simulink model "TB28_A25R_Charging_Stop"  (R2025a)
settings: Solver=FixedStepDiscrete  StartTime=0  StopTime=TB.t_end  FixedStep=TB.dt  RelTol=1e-3
InitFcn:
  | % 모델과 같은 폴더의 초기화 스크립트를 실행해 P(설계 파라미터)와 TB(시험 조건)를 만든다.
  | run(fullfile(fileparts(get_param(bdroot, 'FileName')), 'TB28_init.m'));
values from neighbouring files (symbols this model uses):
  TB = struct()    [TB28_init.m]    (also in run_TB28.m = evalin('base', 'TB'))
libraries: fl_lib x220, nesl_utility x81
(part 1 of 4)
settings Model: Creator=hj000  LastModifiedBy=hj000
settings DataIOCC: SaveOutput=off  SignalLogging=off  SaveTime=off

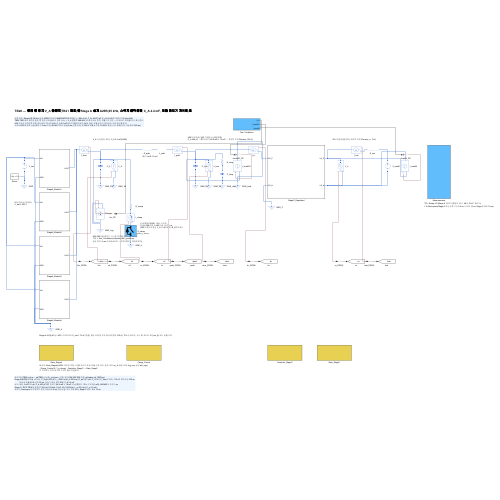
[thumbnail: Simulink's stored preview of the top-level diagram]
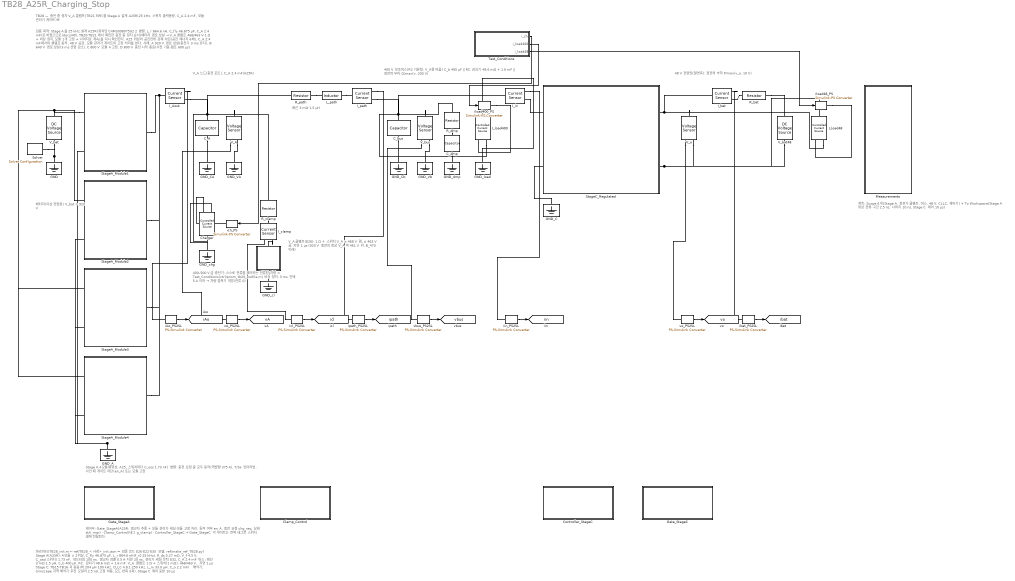
== system TB28_A25R_Charging_Stop ==
  note: TB28 — 충전 중 정지·V_A 클램프(TB21 회로)를 Stage A 설계 A25R(25 kHz, 스위치 출력용량, C_A 2.4 mF, 모듈 관리기 게이트)로
  note: 검증 목적: Stage A를 25 kHz 설계 A25R(위치당 C4MS008075U2 2병렬, L_r 864.6 nH, C_fly 46.875 µF, C_A 2.4 mF)로 바꿨으므로(docs/40),
      | TB20·TB21에서 확인한 충전 중 정지 순서(배터리 경로 상실 → V_A 클램프 468/463 V·1 Ω + 비상 정지, 모듈 1개 고장 → 나머지로 계속)를 다시 확인한다.
      | A25 위상의 공진전류 강제 차단(공진 에너지 6배), C_A 2.4 mF에서의 클램프 동작, 48 V 공급, 모듈 관리기 게이트의 고장 처리를 본다.
      | 사례: A 920 V 경로 상실(충전기 3 ms 유지), B 640 V 경로 상실(3 ms 선형 감소), C 800 V 모듈 4 고장, D 800 V 충전 시작·종료(사전 기동·램프 600 µs)
  note: 배터리(이상 전압원)
      | V_bat = 920 V
  note: V_A 노드(충전 포트), C_A 2.4 mF(A25R)
  note: 400–500 V급 충전기: 스스로 전류를 제어하는 전류원
      | 지령 = Test_Conditions(ctrl/prism_tb20_profile.m)
      | 비상 정지: 3 ms 안에 5 A 이하 → 차량 접촉기 개방(전류 0)
  note: V_A 클램프(E26): 1 Ω + 스위치
      | V_A ≥ 468 V 켬, ≤ 463 V 끔, 지연 1 µs
      | (920 V 충전의 정상 V_A 약 461 V 위, B_470 아래)
  note: Stage A 4모듈(8위상, A25, 스위치마다 C_oss 1.73 nF) 병렬: 충전 요청 중 모두 동작(역방향 375 A), T/16 인터리빙. 사건 때 게이트 차단(en_A) 또는 모듈 고장
  note: 배선 3 mΩ·1.5 µH
  note: 400 V 보조버스(R2 기본형: V_A를 따름)
      | C_b 400 µF ∥ RC 감쇠기 48.6 mΩ + 1.6 mF ∥ 정전력 부하 Q/max(v, 200 V)
  note: 48 V 전원망(절연측): 정전력 부하 P/max(v_o, 10 V)
  note: 제어부: Gate_StageA(A25R: 영교차 추종 + 모듈 관리기·셰딩·모듈 고장 처리, 동작 여부 en_A, 충전 요청 chg_req, 상태 stA_mgr)
      | · Clamp_Control(태그 g_clamp) · Controller_StageC → Gate_StageC
      | 각 게이트는 전역 태그로 스위치 셀에 전달된다.
  note: 계측: Scope 6개(Stage A, 충전기·클램프, 버스, 48 V, CLLC, 제어기)
      | + To Workspace(Stage A 위상 전류·구간 2.5 ns, 나머지 10 ns, Stage C 제어 10 µs)
  note: 파라미터(TB28_init.m ← ref/TB28_<사례>_init.json = 검증 코드 E26·E22·E35 모델, ref/make_ref_TB28.py)
      | Stage A(A25R): 4모듈 × 2위상, C_fly 46.875 µF, L_r 864.6 nH(f_r0 25 kHz), R_ds 5.27 mΩ, V_f 4.5 V, C_oss(스위치) 1.73 nF, 데드타임 100 ns,
      |          영교차 검출 0.5 A·지연 20 ns, 관리기·셰딩 문턱 E32, C_A 2.4 mF
      | 버스: 배선 3 mΩ·1.5 µH, C_b 400 µF, RC 감쇠기 48.6 mΩ + 1.6 mF. V_A 클램프 1 Ω + 스위치(1 mΩ), 468/463 V, 지연 1 µs
      | Stage C: TB15·TB16과 같음(벅 204 µH·100 kHz, CLLC 4.8:1·250 kHz, L_m 33.0 µH, C_o 2.2 mF)
      | 해석기: Simscape 지역 해석기 후진 오일러 2.5 ns(고정 비용, 모드 반복 3회), Stage C 제어 표본 10 µs
  C_A : fl_lib/Electrical/Electrical Elements/Capacitor  c=TB.A.CA F  r=1e-6 Ohm  g=0 1/Ohm  i_specify=off  i_priority=None  i=0 A  i_nominal_specify=off  i_nominal_value=1  i_nominal_unit=A  v_specify=off  v_priority=None  v=0 V  v_nominal_specify=off  v_nominal_value=1  v_nominal_unit=V  vc_specify=on  vc_priority=High  vc=TB.vA0 V  vc_nominal_specify=off  vc_nominal_value=1  vc_nominal_unit=V
  C_bus : fl_lib/Electrical/Electrical Elements/Capacitor  c=TB.Cb F  r=1e-6 Ohm  g=0 1/Ohm  i_specify=off  i_priority=None  i=0 A  i_nominal_specify=off  i_nominal_value=1  i_nominal_unit=A  v_specify=off  v_priority=None  v=0 V  v_nominal_specify=off  v_nominal_value=1  v_nominal_unit=V  vc_specify=on  vc_priority=High  vc=TB.vb0 V  vc_nominal_specify=off  vc_nominal_value=1  vc_nominal_unit=V
  C_dmp : fl_lib/Electrical/Electrical Elements/Capacitor  c=TB.Cdmp F  r=1e-6 Ohm  g=0 1/Ohm  i_specify=off  i_priority=None  i=0 A  i_nominal_specify=off  i_nominal_value=1  i_nominal_unit=A  v_specify=off  v_priority=None  v=0 V  v_nominal_specify=off  v_nominal_value=1  v_nominal_unit=V  vc_specify=on  vc_priority=High  vc=TB.vb0 V  vc_nominal_specify=off  vc_nominal_value=1  vc_nominal_unit=V
  Charger : fl_lib/Electrical/Electrical Sources/Controlled Current Source
  Clamp_Control : Subsystem
  Controller_StageC : Subsystem
  GND : fl_lib/Electrical/Electrical Elements/Electrical Reference
  GND_A : fl_lib/Electrical/Electrical Elements/Electrical Reference
  GND_C : fl_lib/Electrical/Electrical Elements/Electrical Reference
  GND_CA : fl_lib/Electrical/Electrical Elements/Electrical Reference
  GND_Cb : fl_lib/Electrical/Electrical Elements/Electrical Reference
  GND_VA : fl_lib/Electrical/Electrical Elements/Electrical Reference
  GND_Vb : fl_lib/Electrical/Electrical Elements/Electrical Reference
  GND_chg : fl_lib/Electrical/Electrical Elements/Electrical Reference
  GND_cl : fl_lib/Electrical/Electrical Elements/Electrical Reference
  GND_dmp : fl_lib/Electrical/Electrical Elements/Electrical Reference
  GND_load : fl_lib/Electrical/Electrical Elements/Electrical Reference
  Gate_StageA : Subsystem
  Gate_StageC : Subsystem
  I_Aout : fl_lib/Electrical/Electrical Sensors/Current Sensor
  I_bat : fl_lib/Electrical/Electrical Sensors/Current Sensor
  I_clamp : fl_lib/Electrical/Electrical Sensors/Current Sensor
  I_in : fl_lib/Electrical/Electrical Sensors/Current Sensor
  I_load400 : fl_lib/Electrical/Electrical Sources/Controlled Current Source
  I_load48 : fl_lib/Electrical/Electrical Sources/Controlled Current Source
  I_path : fl_lib/Electrical/Electrical Sensors/Current Sensor
  L_path : fl_lib/Electrical/Electrical Elements/Inductor  l=TB.Lpath H  r=0 Ohm  g=1e-9 1/Ohm  i_specify=off  i_priority=None  i=0 A  i_nominal_specify=off  i_nominal_value=1  i_nominal_unit=A  v_specify=off  v_priority=None  v=0 V  v_nominal_specify=off  v_nominal_value=1  v_nominal_unit=V  i_L_specify=on  i_L_priority=High  i_L=TB.iw0 A  i_L_nominal_specify=off  i_L_nominal_value=1  i_L_nominal_unit=A
  Measurements : Subsystem
  R_bat : fl_lib/Electrical/Electrical Elements/Resistor  R=TB.Rbat Ohm  i_specify=off  i_priority=None  i=0 A  i_nominal_specify=off  i_nominal_value=1  i_nominal_unit=A  v_specify=off  v_priority=None  v=0 V  v_nominal_specify=off  v_nominal_value=1  v_nominal_unit=V
  R_clamp : fl_lib/Electrical/Electrical Elements/Resistor  R=TB.Rclamp Ohm  i_specify=off  i_priority=None  i=0 A  i_nominal_specify=off  i_nominal_value=1  i_nominal_unit=A  v_specify=off  v_priority=None  v=0 V  v_nominal_specify=off  v_nominal_value=1  v_nominal_unit=V
  R_dmp : fl_lib/Electrical/Electrical Elements/Resistor  R=TB.Rdmp Ohm  i_specify=off  i_priority=None  i=0 A  i_nominal_specify=off  i_nominal_value=1  i_nominal_unit=A  v_specify=off  v_priority=None  v=0 V  v_nominal_specify=off  v_nominal_value=1  v_nominal_unit=V
  R_path : fl_lib/Electrical/Electrical Elements/Resistor  R=TB.Rpath Ohm  i_specify=off  i_priority=None  i=0 A  i_nominal_specify=off  i_nominal_value=1  i_nominal_unit=A  v_specify=off  v_priority=None  v=0 V  v_nominal_specify=off  v_nominal_value=1  v_nominal_unit=V
  S_clamp : Subsystem  mask(PRISM-Hub switch cell){Ron=1e-3, Goff=1e-8, Vf=2, Rd=1e-3, Goffd=1e-8}
      mask prompts: Ron "도통 저항 R_on [Ohm]"; Goff "차단 컨덕턴스 G_off [S]"; Vf "다이오드 순방향 전압 Vf [V]"; Rd "다이오드 도통 저항 R_d [Ohm]"; Goffd "다이오드 차단 컨덕턴스 [S]"
      mask help: 전력 반도체 스위치 셀 S_clamp. 게이트 태그 g_clamp.
      settings: AttributesFormatString=gate: g_clamp
      mask Display:
      | plot([0.50 0.50 ],[0.95 0.65 ],[0.50 0.74 ],[0.65 0.35 ],[0.50 0.50 ],[0.35 0.05 ]);
      | plot([0.50 0.20 0.20 ],[0.80 0.80 0.58 ],[0.20 0.20 0.50 ],[0.42 0.20 0.20 ]);
      | plot([0.20 0.10 0.30 0.20 ],[0.58 0.42 0.42 0.58 ],[0.10 0.30 ],[0.58 0.58 ]);
      | port_label('LConn',1,'D');
      | port_label('RConn',1,'S');
  Solver : nesl_utility/Solver Configuration  PhysicalDomain=network_engine_domain  SubClassName=solver  LeftPortType=input  RightPortType=generic  Tones=[]  Harmonics=[]  SimulateNoise=off  Profile=off  UseLocalSampling=off  EnableSwitchedLinearOptims=on  FrequencyDomain=off  UseCCode=off  RelTol=0.001  AbsTol=0.001  MinStep=1e-09  ToWorkspace=off  RevertToSquareIcSolve=off  NumHomotopyIterations=100  PhasorMode=off  PhasorModeNumHarmonics=1  ConsistencySolver=NEWTON_XTOL_AFTER_FTOL  IndexReductionMethod=DerivativeReplacement  DoDC=off  ResidualTolerance=1e-9  ConsistencyTolSource=GLOBAL  ConsistencyAbsTol=0.001  ConsistencyRelTol=0.001  ConsistencyTolFactor=0.001  UseLocalSolver=on  LocalSolverChoice=NE_BACKWARD_EULER_ADVANCER  ResolveIndetEquations=on  FunctionEvalNumThread=1  LocalSolverSampleTime=TB.dt  DoFixedCost=on  MaxNonlinIter=3  MaxModeIter=2  ComputeImpulses=off  ImpulseIterations=2  LinearAlgebra=auto  LinearAlgebraNumThread=0  EquationFormulation=NE_TIME_EF  DelaysMemoryBudget=1024  AutomaticFiltering=on  FilteringTimeConstant=0.001  PartitionStorageMethod=AS_NEEDED  PartitionMemoryBudget=1024  PartitionMethod=ROBUST  MultibodyUseLocalSolver=off  MultibodyLocalSolverChoice=ODE1  MultibodyLocalSolverSampleTime=0.001
  StageA_Module1 : Subsystem
  StageA_Module2 : Subsystem
  StageA_Module3 : Subsystem
  StageA_Module4 : Subsystem
  StageC_Regulated : Subsystem
  Test_Conditions : Subsystem
  V_A : fl_lib/Electrical/Electrical Sensors/Voltage Sensor
  V_bat : fl_lib/Electrical/Electrical Sources/DC Voltage Source  v0=TB.vbat V
  V_bat48 : fl_lib/Electrical/Electrical Sources/DC Voltage Source  v0=TB.OCV V
  V_bus : fl_lib/Electrical/Electrical Sensors/Voltage Sensor
  V_o : fl_lib/Electrical/Electrical Sensors/Voltage Sensor
  iAo_PS2SL : nesl_utility/PS-Simulink Converter  PhysicalDomain=network_engine_domain  SubClassName=ps_output  LeftPortType=input  RightPortType=output  PseudoPeriodic=off  Frequencies=[]  VectorFormat=inherit  Unit=inherit  AffineConversion=off
  ibat_PS2SL : nesl_utility/PS-Simulink Converter  PhysicalDomain=network_engine_domain  SubClassName=ps_output  LeftPortType=input  RightPortType=output  PseudoPeriodic=off  Frequencies=[]  VectorFormat=inherit  Unit=inherit  AffineConversion=off
  ich_PS : nesl_utility/Simulink-PS Converter  PhysicalDomain=network_engine_domain  SubClassName=ps_input  LeftPortType=input  RightPortType=output  PseudoPeriodic=off  Frequencies=[]  NoiseDistribution=none  NoiseParameters=[]  Unit=1  AffineConversion=off  FilteringAndDerivatives=provide  SimscapeFilterOrder=1  InputFilterTimeConstant=0.001  UdotUserProvided=0
  icl_PS2SL : nesl_utility/PS-Simulink Converter  PhysicalDomain=network_engine_domain  SubClassName=ps_output  LeftPortType=input  RightPortType=output  PseudoPeriodic=off  Frequencies=[]  VectorFormat=inherit  Unit=inherit  AffineConversion=off
  iin_PS2SL : nesl_utility/PS-Simulink Converter  PhysicalDomain=network_engine_domain  SubClassName=ps_output  LeftPortType=input  RightPortType=output  PseudoPeriodic=off  Frequencies=[]  VectorFormat=inherit  Unit=inherit  AffineConversion=off
  iload400_PS : nesl_utility/Simulink-PS Converter  PhysicalDomain=network_engine_domain  SubClassName=ps_input  LeftPortType=input  RightPortType=output  PseudoPeriodic=off  Frequencies=[]  NoiseDistribution=none  NoiseParameters=[]  Unit=1  AffineConversion=off  FilteringAndDerivatives=provide  SimscapeFilterOrder=1  InputFilterTimeConstant=0.001  UdotUserProvided=0
  iload48_PS : nesl_utility/Simulink-PS Converter  PhysicalDomain=network_engine_domain  SubClassName=ps_input  LeftPortType=input  RightPortType=output  PseudoPeriodic=off  Frequencies=[]  NoiseDistribution=none  NoiseParameters=[]  Unit=1  AffineConversion=off  FilteringAndDerivatives=provide  SimscapeFilterOrder=1  InputFilterTimeConstant=0.001  UdotUserProvided=0
  ipath_PS2SL : nesl_utility/PS-Simulink Converter  PhysicalDomain=network_engine_domain  SubClassName=ps_output  LeftPortType=input  RightPortType=output  PseudoPeriodic=off  Frequencies=[]  VectorFormat=inherit  Unit=inherit  AffineConversion=off
  vA_PS2SL : nesl_utility/PS-Simulink Converter  PhysicalDomain=network_engine_domain  SubClassName=ps_output  LeftPortType=input  RightPortType=output  PseudoPeriodic=off  Frequencies=[]  VectorFormat=inherit  Unit=inherit  AffineConversion=off
  vbus_PS2SL : nesl_utility/PS-Simulink Converter  PhysicalDomain=network_engine_domain  SubClassName=ps_output  LeftPortType=input  RightPortType=output  PseudoPeriodic=off  Frequencies=[]  VectorFormat=inherit  Unit=inherit  AffineConversion=off
  vo_PS2SL : nesl_utility/PS-Simulink Converter  PhysicalDomain=network_engine_domain  SubClassName=ps_output  LeftPortType=input  RightPortType=output  PseudoPeriodic=off  Frequencies=[]  VectorFormat=inherit  Unit=inherit  AffineConversion=off
  tag scope: iAo=global, ibat=global, icl=global, iin=global, ipath=global, vA=global, vbus=global, vo=global
  wires:
  iAo_PS2SL/1 -> [iAo]
  vA_PS2SL/1 -> [vA]
  icl_PS2SL/1 -> [icl]
  ipath_PS2SL/1 -> [ipath]
  vbus_PS2SL/1 -> [vbus]
  iin_PS2SL/1 -> [iin]
  vo_PS2SL/1 -> [vo]
  ibat_PS2SL/1 -> [ibat]
  Test_Conditions/1(i_ch) -> ich_PS/1
  Test_Conditions/2(i_load400) -> iload400_PS/1
  Test_Conditions/3(i_load48) -> iload48_PS/1
  connections:
  GND/LConn1 -- Solver/RConn1 -- V_bat/RConn1
  StageA_Module1/LConn1 -- V_bat/LConn1 -- StageA_Module2/LConn1 -- StageA_Module3/LConn1 -- StageA_Module4/LConn1
  StageA_Module1/LConn2 -- StageA_Module2/LConn2 -- StageA_Module3/LConn2 -- GND_A/LConn1 -- StageA_Module4/LConn2
  StageA_Module1/RConn1 -- StageA_Module2/RConn1 -- StageA_Module3/RConn1 -- I_Aout/LConn1 -- StageA_Module4/RConn1
  I_Aout/RConn2 -- V_A/LConn1 -- Charger/LConn1 -- R_clamp/LConn1 -- C_A/LConn1 -- R_path/LConn1
  C_A/RConn1 -- GND_CA/LConn1
  V_A/RConn2 -- GND_VA/LConn1
  Charger/RConn2 -- GND_chg/LConn1
  ich_PS/RConn1 -- Charger/RConn1
  R_clamp/RConn1 -- I_clamp/LConn1
  I_clamp/RConn2 -- S_clamp/LConn1
  S_clamp/RConn1 -- GND_cl/LConn1
  R_path/RConn1 -- L_path/LConn1
  L_path/RConn1 -- I_path/LConn1
  I_path/RConn2 -- V_bus/LConn1 -- R_dmp/LConn1 -- I_load400/RConn2 -- C_bus/LConn1 -- I_in/LConn1
  C_bus/RConn1 -- GND_Cb/LConn1
  V_bus/RConn2 -- GND_Vb/LConn1
  R_dmp/RConn1 -- C_dmp/LConn1
  C_dmp/RConn1 -- GND_dmp/LConn1
  I_load400/LConn1 -- GND_load/LConn1
  iload400_PS/RConn1 -- I_load400/RConn1
  I_in/RConn2 -- StageC_Regulated/LConn1
  StageC_Regulated/LConn2 -- GND_C/LConn1
  V_o/LConn1 -- I_bat/LConn1 -- StageC_Regulated/RConn1 -- I_load48/RConn2
  V_o/RConn2 -- V_bat48/RConn1 -- StageC_Regulated/RConn2 -- I_load48/LConn1
  I_bat/RConn2 -- R_bat/LConn1
  R_bat/RConn1 -- V_bat48/LConn1
  iload48_PS/RConn1 -- I_load48/RConn1
  I_Aout/RConn1 -- iAo_PS2SL/LConn1
  V_A/RConn1 -- vA_PS2SL/LConn1
  I_clamp/RConn1 -- icl_PS2SL/LConn1
  I_path/RConn1 -- ipath_PS2SL/LConn1
  V_bus/RConn1 -- vbus_PS2SL/LConn1
  I_in/RConn1 -- iin_PS2SL/LConn1
  V_o/RConn1 -- vo_PS2SL/LConn1
  I_bat/RConn1 -- ibat_PS2SL/LConn1

== system TB28_A25R_Charging_Stop/Clamp_Control ==
  note: V_A 클램프 비교기(ctrl/prism_va_clamp.m, 검증 코드 E26과 같은 논리): V_A ≥ v_on 켬, ≤ v_off 끔(켜진 동안 v_A > v_off이면 유지),
      | 요청이 n_delay 간격(1 µs) 이어지면 상태를 바꾼다. 측정은 한 간격 지연과 시작 표본 보호를 거친다.
  Clock : DigitalClock  SampleTime=TB.dt
  Startup_guard : Switch  Threshold=TB.guard_t  SaturateOnIntegerOverflow=off  InputSameDT=off
  Startup_guard_init : Constant  Value=TB.vA0
  VA_Clamp : MATLAB Function  TreatAsAtomicUnit=on
  clamp_prm : Constant  Value=TB.clamp_prm
  vA_z1 : UnitDelay  InitialCondition=TB.vA0  SampleTime=TB.dt  HasFrameUpgradeWarning=on
  tag scope: clamp_st=global, g_clamp=global
  wires:
  [vA] -> vA_z1/1
  Startup_guard_init/1 -> Startup_guard/3
  vA_z1/1 -> Startup_guard/1
  Clock/1 -> Startup_guard/2, VA_Clamp/1(t)
  Startup_guard/1 -> VA_Clamp/2(vA)
  clamp_prm/1 -> VA_Clamp/3(prm)
  VA_Clamp/1(g) -> [g_clamp]
  VA_Clamp/2(st_out) -> [clamp_st]

== system TB28_A25R_Charging_Stop/Controller_StageC ==
  note: 조정형 Stage C 제어기(검증 코드 E22 control과 같은 알고리즘·게인, 표본 10 µs, 계산 지연 1주기, TB16과 같음)
      | 전류 PI 적분은 평형값에서 시작(prm(27), TB17과 같음). 입력 v_bus는 실제 버스.
  Clock : DigitalClock  SampleTime=TB.dt
  StageC_Controller : MATLAB Function  TreatAsAtomicUnit=on
  Startup_guard : Switch  Threshold=TB.guard_t  SaturateOnIntegerOverflow=off  InputSameDT=off
  Startup_guard_init : Constant  Value=TB.meas0
  ctl_prm : Constant  Value=TB.ctl_prm
  meas_mux : Mux  Inputs=6
  meas_z1 : UnitDelay  InitialCondition=TB.meas0  SampleTime=TB.dt  HasFrameUpgradeWarning=on
  tag scope: ucC=global
  wires:
  [vbus] -> meas_mux/1
  [iL] -> meas_mux/2
  [vI] -> meas_mux/3
  [vo] -> meas_mux/4
  [iload] -> meas_mux/5
  [ibat] -> meas_mux/6
  meas_mux/1 -> meas_z1/1
  Startup_guard_init/1 -> Startup_guard/3
  meas_z1/1 -> Startup_guard/1
  Clock/1 -> Startup_guard/2, StageC_Controller/1(t)
  Startup_guard/1 -> StageC_Controller/2(meas)
  ctl_prm/1 -> StageC_Controller/3(prm)
  StageC_Controller/1(u) -> [ucC]

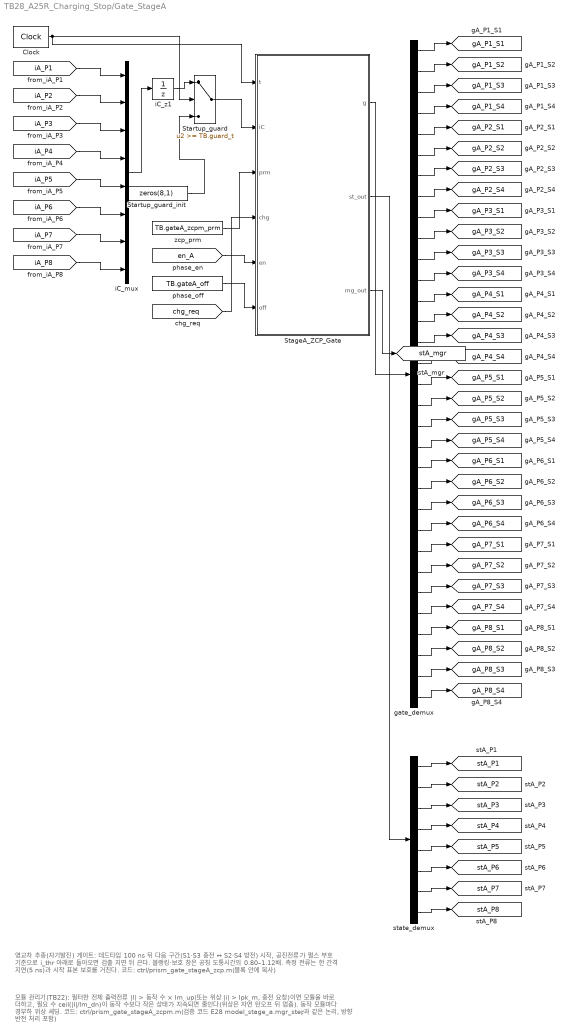
== system TB28_A25R_Charging_Stop/Gate_StageA ==
  note: 모듈 관리기(TB22): 필터한 전체 출력전류 |I| > 동작 수 × Im_up(또는 위상 |i| > Ipk_m, 충전 요청)이면 모듈을 바로 더하고,
      | 필요 수 ceil(|I|/Im_dn)이 동작 수보다 작은 상태가 지속되면 줄인다(위상은 자연 턴오프 뒤 멈춤). 동작 모듈마다 경부하 위상 셰딩.
      | 코드: ctrl/prism_gate_stageA_zcpm.m(검증 코드 E28 model_stage_a.mgr_step과 같은 논리, 방향 반전 처리 포함)
  note: 영교차 추종(자기발진) 게이트: 데드타임 100 ns 뒤 다음 구간(S1·S3 충전 ↔ S2·S4 방전) 시작,
      | 공진전류가 펄스 부호 기준으로 i_thr 아래로 돌아오면 검출 지연 뒤 끈다. 블랭킹·보호 창은 공칭 도통시간의 0.80–1.12배.
      | 측정 전류는 한 간격 지연(5 ns)과 시작 표본 보호를 거친다. 코드: ctrl/prism_gate_stageA_zcp.m(블록 안에 복사)
  Clock : DigitalClock  SampleTime=TB.dt
  StageA_ZCP_Gate : MATLAB Function  TreatAsAtomicUnit=on
  Startup_guard : Switch  Threshold=TB.guard_t  SaturateOnIntegerOverflow=off  InputSameDT=off
  Startup_guard_init : Constant  Value=zeros(8,1)
  gate_demux : Demux  Outputs=[1 1 1 1 1 1 1 1 1 1 1 1 1 1 1 1 1 1 1 1 1 1 1 1 1 1 1 1 1 1 1 1]
  iC_mux : Mux  Inputs=8
  iC_z1 : UnitDelay  SampleTime=TB.dt  HasFrameUpgradeWarning=on
  phase_off : Constant  Value=TB.gateA_off
  state_demux : Demux  Outputs=[1 1 1 1 1 1 1 1]
  zcp_prm : Constant  Value=TB.gateA_zcpm_prm
  tag scope: gA_P1_S1=global, gA_P1_S2=global, gA_P1_S3=global, gA_P1_S4=global, gA_P2_S1=global, gA_P2_S2=global, gA_P2_S3=global, gA_P2_S4=global, gA_P3_S1=global, gA_P3_S2=global, gA_P3_S3=global, gA_P3_S4=global, gA_P4_S1=global, gA_P4_S2=global, gA_P4_S3=global, gA_P4_S4=global, gA_P5_S1=global, gA_P5_S2=global, gA_P5_S3=global, gA_P5_S4=global, gA_P6_S1=global, gA_P6_S2=global, gA_P6_S3=global, gA_P6_S4=global, gA_P7_S1=global, gA_P7_S2=global, gA_P7_S3=global, gA_P7_S4=global, gA_P8_S1=global, gA_P8_S2=global, gA_P8_S3=global, gA_P8_S4=global, stA_P1=global, stA_P2=global, stA_P3=global, stA_P4=global, stA_P5=global, stA_P6=global, stA_P7=global, stA_P8=global, stA_mgr=global
  wires:
  [iA_P1] -> iC_mux/1
  [iA_P2] -> iC_mux/2
  [iA_P3] -> iC_mux/3
  [iA_P4] -> iC_mux/4
  [iA_P5] -> iC_mux/5
  [iA_P6] -> iC_mux/6
  [iA_P7] -> iC_mux/7
  [iA_P8] -> iC_mux/8
  iC_mux/1 -> iC_z1/1
  Startup_guard_init/1 -> Startup_guard/3
  iC_z1/1 -> Startup_guard/1
  Clock/1 -> Startup_guard/2, StageA_ZCP_Gate/1(t)
  StageA_ZCP_Gate/3(mg_out) -> [stA_mgr]
  Startup_guard/1 -> StageA_ZCP_Gate/2(iC)
  zcp_prm/1 -> StageA_ZCP_Gate/3(prm)
  [chg_req] -> StageA_ZCP_Gate/4(chg)
  [en_A] -> StageA_ZCP_Gate/5(en)
  phase_off/1 -> StageA_ZCP_Gate/6(off)
  StageA_ZCP_Gate/1(g) -> gate_demux/1
  gate_demux/1 -> [gA_P1_S1]
  gate_demux/2 -> [gA_P1_S2]
  gate_demux/3 -> [gA_P1_S3]
  gate_demux/4 -> [gA_P1_S4]
  gate_demux/5 -> [gA_P2_S1]
  gate_demux/6 -> [gA_P2_S2]
  gate_demux/7 -> [gA_P2_S3]
  gate_demux/8 -> [gA_P2_S4]
  gate_demux/9 -> [gA_P3_S1]
  gate_demux/10 -> [gA_P3_S2]
  gate_demux/11 -> [gA_P3_S3]
  gate_demux/12 -> [gA_P3_S4]
  gate_demux/13 -> [gA_P4_S1]
  gate_demux/14 -> [gA_P4_S2]
  gate_demux/15 -> [gA_P4_S3]
  gate_demux/16 -> [gA_P4_S4]
  gate_demux/17 -> [gA_P5_S1]
  gate_demux/18 -> [gA_P5_S2]
  gate_demux/19 -> [gA_P5_S3]
  gate_demux/20 -> [gA_P5_S4]
  gate_demux/21 -> [gA_P6_S1]
  gate_demux/22 -> [gA_P6_S2]
  gate_demux/23 -> [gA_P6_S3]
  gate_demux/24 -> [gA_P6_S4]
  gate_demux/25 -> [gA_P7_S1]
  gate_demux/26 -> [gA_P7_S2]
  gate_demux/27 -> [gA_P7_S3]
  gate_demux/28 -> [gA_P7_S4]
  gate_demux/29 -> [gA_P8_S1]
  gate_demux/30 -> [gA_P8_S2]
  gate_demux/31 -> [gA_P8_S3]
  gate_demux/32 -> [gA_P8_S4]
  StageA_ZCP_Gate/2(st_out) -> state_demux/1
  state_demux/1 -> [stA_P1]
  state_demux/2 -> [stA_P2]
  state_demux/3 -> [stA_P3]
  state_demux/4 -> [stA_P4]
  state_demux/5 -> [stA_P5]
  state_demux/6 -> [stA_P6]
  state_demux/7 -> [stA_P7]
  state_demux/8 -> [stA_P8]

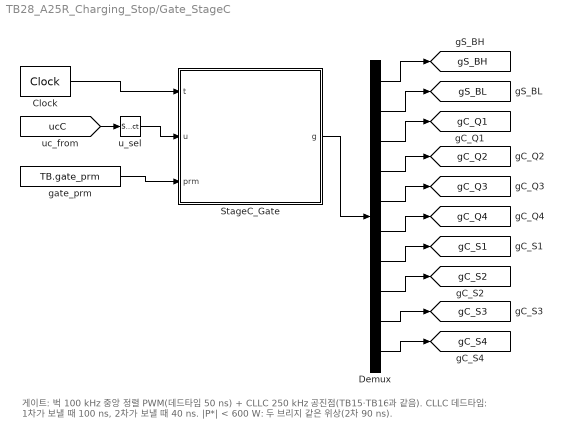
== system TB28_A25R_Charging_Stop/Gate_StageC ==
  note: 게이트: 벅 100 kHz 중앙 정렬 PWM(데드타임 50 ns) + CLLC 250 kHz 공진점(TB15·TB16과 같음).
      | CLLC 데드타임: 1차가 보낼 때 100 ns, 2차가 보낼 때 40 ns. |P*| < 600 W: 두 브리지 같은 위상(2차 90 ns).
  Clock : DigitalClock  SampleTime=TB.dt
  Demux : Demux  Outputs=10
  StageC_Gate : MATLAB Function  TreatAsAtomicUnit=on
  gate_prm : Constant  Value=TB.gate_prm
  u_sel : Selector  InputPortWidth=4  IndexOptions=Index vector (dialog)  Indices=[1 2]  OutputSizes=1
  tag scope: gC_Q1=global, gC_Q2=global, gC_Q3=global, gC_Q4=global, gC_S1=global, gC_S2=global, gC_S3=global, gC_S4=global, gS_BH=global, gS_BL=global
  wires:
  [ucC] -> u_sel/1
  Clock/1 -> StageC_Gate/1(t)
  u_sel/1 -> StageC_Gate/2(u)
  gate_prm/1 -> StageC_Gate/3(prm)
  StageC_Gate/1(g) -> Demux/1
  Demux/1 -> [gS_BH]
  Demux/2 -> [gS_BL]
  Demux/3 -> [gC_Q1]
  Demux/4 -> [gC_Q2]
  Demux/5 -> [gC_Q3]
  Demux/6 -> [gC_Q4]
  Demux/7 -> [gC_S1]
  Demux/8 -> [gC_S2]
  Demux/9 -> [gC_S3]
  Demux/10 -> [gC_S4]

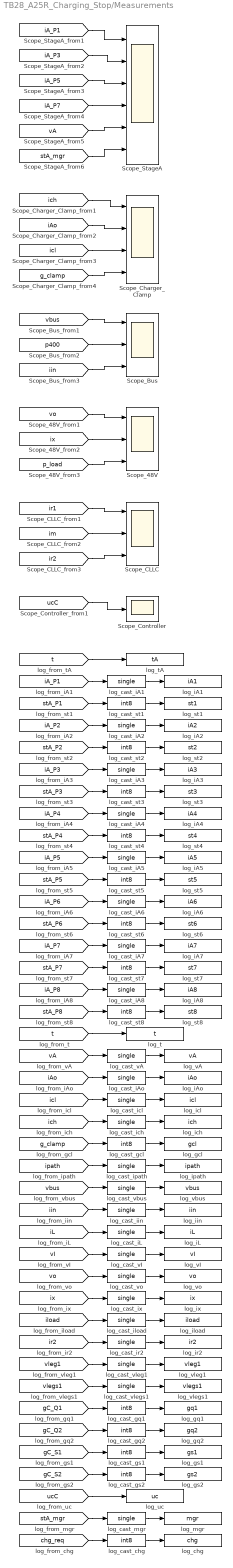
== system TB28_A25R_Charging_Stop/Measurements ==
  Scope_48V : Scope  NumInputPorts=3
      settings: Title=Scope 48V
  Scope_Bus : Scope  NumInputPorts=3
      settings: Title=Scope Bus
  Scope_CLLC : Scope  NumInputPorts=3
      settings: Title=Scope CLLC
  Scope_Charger_Clamp : Scope  NumInputPorts=4
      settings: Title=Scope Charger Clamp
  Scope_Controller : Scope
      settings: Title=Scope Controller
  Scope_StageA : Scope  NumInputPorts=6
      settings: Title=Scope StageA
  log_cast_chg : DataTypeConversion  OutDataTypeStr=int8  SaturateOnIntegerOverflow=off  RndMeth=Floor
  log_cast_gcl : DataTypeConversion  OutDataTypeStr=int8  SaturateOnIntegerOverflow=off  RndMeth=Floor
  log_cast_gq1 : DataTypeConversion  OutDataTypeStr=int8  SaturateOnIntegerOverflow=off  RndMeth=Floor
  log_cast_gq2 : DataTypeConversion  OutDataTypeStr=int8  SaturateOnIntegerOverflow=off  RndMeth=Floor
  log_cast_gs1 : DataTypeConversion  OutDataTypeStr=int8  SaturateOnIntegerOverflow=off  RndMeth=Floor
  log_cast_gs2 : DataTypeConversion  OutDataTypeStr=int8  SaturateOnIntegerOverflow=off  RndMeth=Floor
  log_cast_iA{1..8} (8 alike) : DataTypeConversion  OutDataTypeStr=single  SaturateOnIntegerOverflow=off  RndMeth=Floor
  log_cast_iAo : DataTypeConversion  OutDataTypeStr=single  SaturateOnIntegerOverflow=off  RndMeth=Floor
  log_cast_iL : DataTypeConversion  OutDataTypeStr=single  SaturateOnIntegerOverflow=off  RndMeth=Floor
  log_cast_ich : DataTypeConversion  OutDataTypeStr=single  SaturateOnIntegerOverflow=off  RndMeth=Floor
  log_cast_icl : DataTypeConversion  OutDataTypeStr=single  SaturateOnIntegerOverflow=off  RndMeth=Floor
  log_cast_iin : DataTypeConversion  OutDataTypeStr=single  SaturateOnIntegerOverflow=off  RndMeth=Floor
  log_cast_iload : DataTypeConversion  OutDataTypeStr=single  SaturateOnIntegerOverflow=off  RndMeth=Floor
  log_cast_ipath : DataTypeConversion  OutDataTypeStr=single  SaturateOnIntegerOverflow=off  RndMeth=Floor
  log_cast_ir2 : DataTypeConversion  OutDataTypeStr=single  SaturateOnIntegerOverflow=off  RndMeth=Floor
  log_cast_ix : DataTypeConversion  OutDataTypeStr=single  SaturateOnIntegerOverflow=off  RndMeth=Floor
  log_cast_mgr : DataTypeConversion  OutDataTypeStr=single  SaturateOnIntegerOverflow=off  RndMeth=Floor
  log_cast_st{1..8} (8 alike) : DataTypeConversion  OutDataTypeStr=int8  SaturateOnIntegerOverflow=off  RndMeth=Floor
  log_cast_vA : DataTypeConversion  OutDataTypeStr=single  SaturateOnIntegerOverflow=off  RndMeth=Floor
  log_cast_vI : DataTypeConversion  OutDataTypeStr=single  SaturateOnIntegerOverflow=off  RndMeth=Floor
  log_cast_vbus : DataTypeConversion  OutDataTypeStr=single  SaturateOnIntegerOverflow=off  RndMeth=Floor
  log_cast_vleg1 : DataTypeConversion  OutDataTypeStr=single  SaturateOnIntegerOverflow=off  RndMeth=Floor
  log_cast_vlegs1 : DataTypeConversion  OutDataTypeStr=single  SaturateOnIntegerOverflow=off  RndMeth=Floor
  log_cast_vo : DataTypeConversion  OutDataTypeStr=single  SaturateOnIntegerOverflow=off  RndMeth=Floor
  log_chg : ToWorkspace  VariableName=chg  SampleTime=-1
      settings: Decimation=4
  log_gcl : ToWorkspace  VariableName=gcl  SampleTime=-1
      settings: Decimation=4
  log_gq1 : ToWorkspace  VariableName=gq1  SampleTime=-1
      settings: Decimation=4
  log_gq2 : ToWorkspace  VariableName=gq2  SampleTime=-1
      settings: Decimation=4
  log_gs1 : ToWorkspace  VariableName=gs1  SampleTime=-1
      settings: Decimation=4
  log_gs2 : ToWorkspace  VariableName=gs2  SampleTime=-1
      settings: Decimation=4
  log_iA1 : ToWorkspace  VariableName=iA1  SampleTime=-1
  log_iA2 : ToWorkspace  VariableName=iA2  SampleTime=-1
  log_iA3 : ToWorkspace  VariableName=iA3  SampleTime=-1
  log_iA4 : ToWorkspace  VariableName=iA4  SampleTime=-1
  log_iA5 : ToWorkspace  VariableName=iA5  SampleTime=-1
  log_iA6 : ToWorkspace  VariableName=iA6  SampleTime=-1
  log_iA7 : ToWorkspace  VariableName=iA7  SampleTime=-1
  log_iA8 : ToWorkspace  VariableName=iA8  SampleTime=-1
  log_iAo : ToWorkspace  VariableName=iAo  SampleTime=-1
      settings: Decimation=4
  log_iL : ToWorkspace  VariableName=iL  SampleTime=-1
      settings: Decimation=4
  log_ich : ToWorkspace  VariableName=ich  SampleTime=-1
      settings: Decimation=4
  log_icl : ToWorkspace  VariableName=icl  SampleTime=-1
      settings: Decimation=4
  log_iin : ToWorkspace  VariableName=iin  SampleTime=-1
      settings: Decimation=4
  log_iload : ToWorkspace  VariableName=iload  SampleTime=-1
      settings: Decimation=4
  log_ipath : ToWorkspace  VariableName=ipath  SampleTime=-1
      settings: Decimation=4
  log_ir2 : ToWorkspace  VariableName=ir2  SampleTime=-1
      settings: Decimation=4
  log_ix : ToWorkspace  VariableName=ix  SampleTime=-1
      settings: Decimation=4
  log_mgr : ToWorkspace  VariableName=mgr  SampleTime=-1
      settings: Decimation=4
  log_st1 : ToWorkspace  VariableName=st1  SampleTime=-1
  log_st2 : ToWorkspace  VariableName=st2  SampleTime=-1
  log_st3 : ToWorkspace  VariableName=st3  SampleTime=-1
  log_st4 : ToWorkspace  VariableName=st4  SampleTime=-1
  log_st5 : ToWorkspace  VariableName=st5  SampleTime=-1
  log_st6 : ToWorkspace  VariableName=st6  SampleTime=-1
  log_st7 : ToWorkspace  VariableName=st7  SampleTime=-1
  log_st8 : ToWorkspace  VariableName=st8  SampleTime=-1
  log_t : ToWorkspace  VariableName=t  SampleTime=-1
      settings: Decimation=4
  log_tA : ToWorkspace  VariableName=tA  SampleTime=-1
  log_uc : ToWorkspace  VariableName=uc  SampleTime=-1
      settings: Decimation=4000
  log_vA : ToWorkspace  VariableName=vA  SampleTime=-1
      settings: Decimation=4
  log_vI : ToWorkspace  VariableName=vI  SampleTime=-1
      settings: Decimation=4
  log_vbus : ToWorkspace  VariableName=vbus  SampleTime=-1
      settings: Decimation=4
  log_vleg1 : ToWorkspace  VariableName=vleg1  SampleTime=-1
      settings: Decimation=4
  log_vlegs1 : ToWorkspace  VariableName=vlegs1  SampleTime=-1
      settings: Decimation=4
  log_vo : ToWorkspace  VariableName=vo  SampleTime=-1
      settings: Decimation=4
  wires:
  [iA_P1] -> Scope_StageA/1
  [iA_P3] -> Scope_StageA/2
  [iA_P5] -> Scope_StageA/3
  [iA_P7] -> Scope_StageA/4
  [vA] -> Scope_StageA/5
  [stA_mgr] -> Scope_StageA/6
  [ich] -> Scope_Charger_Clamp/1
  [iAo] -> Scope_Charger_Clamp/2
  [icl] -> Scope_Charger_Clamp/3
  [g_clamp] -> Scope_Charger_Clamp/4
  [vbus] -> Scope_Bus/1
  [p400] -> Scope_Bus/2
  [iin] -> Scope_Bus/3
  [vo] -> Scope_48V/1
  [ix] -> Scope_48V/2
  [p_load] -> Scope_48V/3
  [ir1] -> Scope_CLLC/1
  [im] -> Scope_CLLC/2
  [ir2] -> Scope_CLLC/3
  [ucC] -> Scope_Controller/1
  [t] -> log_tA/1
  [iA_P1] -> log_cast_iA1/1
  log_cast_iA1/1 -> log_iA1/1
  [stA_P1] -> log_cast_st1/1
  log_cast_st1/1 -> log_st1/1
  [iA_P2] -> log_cast_iA2/1
  log_cast_iA2/1 -> log_iA2/1
  [stA_P2] -> log_cast_st2/1
  log_cast_st2/1 -> log_st2/1
  [iA_P3] -> log_cast_iA3/1
  log_cast_iA3/1 -> log_iA3/1
  [stA_P3] -> log_cast_st3/1
  log_cast_st3/1 -> log_st3/1
  [iA_P4] -> log_cast_iA4/1
  log_cast_iA4/1 -> log_iA4/1
  [stA_P4] -> log_cast_st4/1
  log_cast_st4/1 -> log_st4/1
  [iA_P5] -> log_cast_iA5/1
  log_cast_iA5/1 -> log_iA5/1
  [stA_P5] -> log_cast_st5/1
  log_cast_st5/1 -> log_st5/1
  [iA_P6] -> log_cast_iA6/1
  log_cast_iA6/1 -> log_iA6/1
  [stA_P6] -> log_cast_st6/1
  log_cast_st6/1 -> log_st6/1
  [iA_P7] -> log_cast_iA7/1
  log_cast_iA7/1 -> log_iA7/1
  [stA_P7] -> log_cast_st7/1
  log_cast_st7/1 -> log_st7/1
  [iA_P8] -> log_cast_iA8/1
  log_cast_iA8/1 -> log_iA8/1
  [stA_P8] -> log_cast_st8/1
  log_cast_st8/1 -> log_st8/1
  [t] -> log_t/1
  [vA] -> log_cast_vA/1
  log_cast_vA/1 -> log_vA/1
  [iAo] -> log_cast_iAo/1
  log_cast_iAo/1 -> log_iAo/1
  [icl] -> log_cast_icl/1
  log_cast_icl/1 -> log_icl/1
  [ich] -> log_cast_ich/1
  log_cast_ich/1 -> log_ich/1
  [g_clamp] -> log_cast_gcl/1
  log_cast_gcl/1 -> log_gcl/1
  [ipath] -> log_cast_ipath/1
  log_cast_ipath/1 -> log_ipath/1
  [vbus] -> log_cast_vbus/1
  log_cast_vbus/1 -> log_vbus/1
  [iin] -> log_cast_iin/1
  log_cast_iin/1 -> log_iin/1
  [iL] -> log_cast_iL/1
  log_cast_iL/1 -> log_iL/1
  [vI] -> log_cast_vI/1
  log_cast_vI/1 -> log_vI/1
  [vo] -> log_cast_vo/1
  log_cast_vo/1 -> log_vo/1
  [ix] -> log_cast_ix/1
  log_cast_ix/1 -> log_ix/1
  [iload] -> log_cast_iload/1
  log_cast_iload/1 -> log_iload/1
  [ir2] -> log_cast_ir2/1
  log_cast_ir2/1 -> log_ir2/1
  [vleg1] -> log_cast_vleg1/1
  log_cast_vleg1/1 -> log_vleg1/1
  [vlegs1] -> log_cast_vlegs1/1
  log_cast_vlegs1/1 -> log_vlegs1/1
  [gC_Q1] -> log_cast_gq1/1
  log_cast_gq1/1 -> log_gq1/1
  [gC_Q2] -> log_cast_gq2/1
  log_cast_gq2/1 -> log_gq2/1
  [gC_S1] -> log_cast_gs1/1
  log_cast_gs1/1 -> log_gs1/1
  [gC_S2] -> log_cast_gs2/1
  log_cast_gs2/1 -> log_gs2/1
  [ucC] -> log_uc/1
  [stA_mgr] -> log_cast_mgr/1
  log_cast_mgr/1 -> log_mgr/1
  [chg_req] -> log_cast_chg/1
  log_cast_chg/1 -> log_chg/1

== system TB28_A25R_Charging_Stop/S_clamp ==
  note: 스위치 셀: 이상 스위치(R_on, G_off) + 역병렬 바디 다이오드(Vf, R_d)
      | 게이트: 전역 태그 "g_clamp" (> 0.5 이면 도통)
  D_body : fl_lib/Electrical/Electrical Elements/Diode  Vf=Vf V  Ron=Rd Ohm  Goff=Goffd 1/Ohm  i_specify=off  i_priority=None  i=0 A  i_nominal_specify=off  i_nominal_value=1  i_nominal_unit=A  v_specify=off  v_priority=None  v=0 V  v_nominal_specify=off  v_nominal_value=1  v_nominal_unit=V
  Gate_PS : nesl_utility/Simulink-PS Converter  PhysicalDomain=network_engine_domain  SubClassName=ps_input  LeftPortType=input  RightPortType=output  PseudoPeriodic=off  Frequencies=[]  NoiseDistribution=none  NoiseParameters=[]  Unit=1  AffineConversion=off  FilteringAndDerivatives=zero  SimscapeFilterOrder=1  InputFilterTimeConstant=0.001  UdotUserProvided=0
  SW : fl_lib/Electrical/Electrical Elements/Switch  R_closed=Ron Ohm  G_open=Goff 1/Ohm  Threshold=0.5  i_specify=off  i_priority=None  i=0 A  i_nominal_specify=off  i_nominal_value=1  i_nominal_unit=A  v_specify=off  v_priority=None  v=0 V  v_nominal_specify=off  v_nominal_value=1  v_nominal_unit=V
  D : PMIOPort  Side=Left
  S : PMIOPort  Port=2  Side=Right
  wires:
  [g_clamp] -> Gate_PS/1
  connections:
  Gate_PS/RConn1 -- SW/RConn1
  SW/LConn1 -- D/RConn1 -- D_body/RConn1
  S/RConn1 -- SW/RConn2 -- D_body/LConn1

== system TB28_A25R_Charging_Stop/StageA_Module1 ==
  note: Stage A 모듈 1: 위상 1·2 병렬(목표 정격 37.5 kW)
      | 각 위상은 영교차 추종 게이트로 자기 공진전류가 0일 때 끈다(ZCS). 두 위상은 T/4 엇갈려 시작한다.
  StageA_Phase1 : Subsystem
  StageA_Phase2 : Subsystem
  VIN : PMIOPort  Side=Left
  GND : PMIOPort  Port=2  Side=Left
  VOUT : PMIOPort  Port=3  Side=Right
  connections:
  VIN/RConn1 -- StageA_Phase1/LConn1 -- StageA_Phase2/LConn1
  GND/RConn1 -- StageA_Phase1/LConn2 -- StageA_Phase2/LConn2
  VOUT/RConn1 -- StageA_Phase1/RConn1 -- StageA_Phase2/RConn1

== system TB28_A25R_Charging_Stop/StageA_Module2 ==
  note: Stage A 모듈 2: 위상 3·4 병렬(목표 정격 37.5 kW)
      | 각 위상은 영교차 추종 게이트로 자기 공진전류가 0일 때 끈다(ZCS). 두 위상은 T/4 엇갈려 시작한다.
  StageA_Phase3 : Subsystem
  StageA_Phase4 : Subsystem
  VIN : PMIOPort  Side=Left
  GND : PMIOPort  Port=2  Side=Left
  VOUT : PMIOPort  Port=3  Side=Right
  connections:
  VIN/RConn1 -- StageA_Phase3/LConn1 -- StageA_Phase4/LConn1
  GND/RConn1 -- StageA_Phase3/LConn2 -- StageA_Phase4/LConn2
  VOUT/RConn1 -- StageA_Phase3/RConn1 -- StageA_Phase4/RConn1

== system TB28_A25R_Charging_Stop/StageA_Module3 ==
  note: Stage A 모듈 3: 위상 5·6 병렬(목표 정격 37.5 kW)
      | 각 위상은 영교차 추종 게이트로 자기 공진전류가 0일 때 끈다(ZCS). 두 위상은 T/4 엇갈려 시작한다.
  StageA_Phase5 : Subsystem
  StageA_Phase6 : Subsystem
  VIN : PMIOPort  Side=Left
  GND : PMIOPort  Port=2  Side=Left
  VOUT : PMIOPort  Port=3  Side=Right
  connections:
  VIN/RConn1 -- StageA_Phase5/LConn1 -- StageA_Phase6/LConn1
  GND/RConn1 -- StageA_Phase5/LConn2 -- StageA_Phase6/LConn2
  VOUT/RConn1 -- StageA_Phase5/RConn1 -- StageA_Phase6/RConn1

== system TB28_A25R_Charging_Stop/StageA_Module4 ==
  note: Stage A 모듈 4: 위상 7·8 병렬(목표 정격 37.5 kW)
      | 각 위상은 영교차 추종 게이트로 자기 공진전류가 0일 때 끈다(ZCS). 두 위상은 T/4 엇갈려 시작한다.
  StageA_Phase7 : Subsystem
  StageA_Phase8 : Subsystem
  VIN : PMIOPort  Side=Left
  GND : PMIOPort  Port=2  Side=Left
  VOUT : PMIOPort  Port=3  Side=Right
  connections:
  VIN/RConn1 -- StageA_Phase7/LConn1 -- StageA_Phase8/LConn1
  GND/RConn1 -- StageA_Phase7/LConn2 -- StageA_Phase8/LConn2
  VOUT/RConn1 -- StageA_Phase7/RConn1 -- StageA_Phase8/RConn1

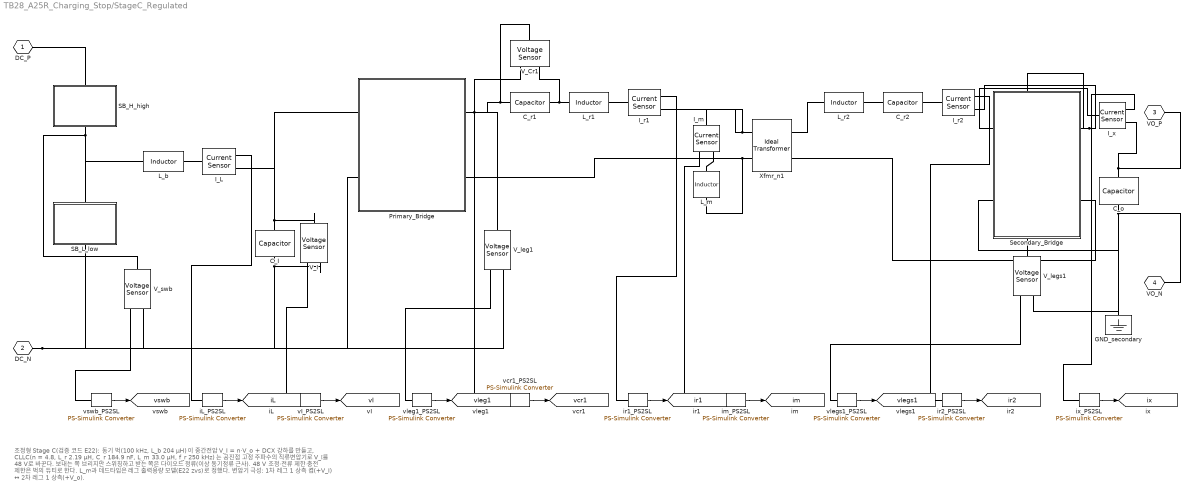
== system TB28_A25R_Charging_Stop/StageC_Regulated ==
  note: 조정형 Stage C(검증 코드 E22): 동기 벅(100 kHz, L_b 204 µH)이 중간전압 V_I = n·V_o + DCX 강하를 만들고,
      | CLLC(n = 4.8, L_r 2.19 µH, C_r 184.9 nF, L_m 33.0 µH, f_r 250 kHz)는 공진점 고정 주파수의 직류변압기로 V_I를 48 V로 바꾼다.
      | 보내는 쪽 브리지만 스위칭하고 받는 쪽은 다이오드 정류(이상 동기정류 근사). 48 V 조정·전류 제한·충전 제한은 벅의 듀티로 한다.
      | L_m과 데드타임은 레그 출력용량 모델(E22 zvs)로 정했다. 변압기 극성: 1차 레그 1 상측 켬(+V_I) ↔ 2차 레그 1 상측(+V_o).
  C_I : fl_lib/Electrical/Electrical Elements/Capacitor  c=TB.C.CI F  r=1e-6 Ohm  g=0 1/Ohm  i_specify=off  i_priority=None  i=0 A  i_nominal_specify=off  i_nominal_value=1  i_nominal_unit=A  v_specify=off  v_priority=None  v=0 V  v_nominal_specify=off  v_nominal_value=1  v_nominal_unit=V  vc_specify=on  vc_priority=High  vc=TB.x0(2) V  vc_nominal_specify=off  vc_nominal_value=1  vc_nominal_unit=V
  C_o : fl_lib/Electrical/Electrical Elements/Capacitor  c=TB.C.Co F  r=1e-6 Ohm  g=0 1/Ohm  i_specify=off  i_priority=None  i=0 A  i_nominal_specify=off  i_nominal_value=1  i_nominal_unit=A  v_specify=off  v_priority=None  v=0 V  v_nominal_specify=off  v_nominal_value=1  v_nominal_unit=V  vc_specify=on  vc_priority=High  vc=TB.x0(3) V  vc_nominal_specify=off  vc_nominal_value=1  vc_nominal_unit=V
  C_r1 : fl_lib/Electrical/Electrical Elements/Capacitor  c=TB.C.Cr1 F  r=1e-6 Ohm  g=0 1/Ohm  i_specify=off  i_priority=None  i=0 A  i_nominal_specify=off  i_nominal_value=1  i_nominal_unit=A  v_specify=off  v_priority=None  v=0 V  v_nominal_specify=off  v_nominal_value=1  v_nominal_unit=V  vc_specify=on  vc_priority=High  vc=0 V  vc_nominal_specify=off  vc_nominal_value=1  vc_nominal_unit=V
  C_r2 : fl_lib/Electrical/Electrical Elements/Capacitor  c=TB.C.Cr2 F  r=1e-6 Ohm  g=0 1/Ohm  i_specify=off  i_priority=None  i=0 A  i_nominal_specify=off  i_nominal_value=1  i_nominal_unit=A  v_specify=off  v_priority=None  v=0 V  v_nominal_specify=off  v_nominal_value=1  v_nominal_unit=V  vc_specify=on  vc_priority=High  vc=0 V  vc_nominal_specify=off  vc_nominal_value=1  vc_nominal_unit=V
  GND_secondary : fl_lib/Electrical/Electrical Elements/Electrical Reference
  I_L : fl_lib/Electrical/Electrical Sensors/Current Sensor
  I_m : fl_lib/Electrical/Electrical Sensors/Current Sensor
  I_r1 : fl_lib/Electrical/Electrical Sensors/Current Sensor
  I_r2 : fl_lib/Electrical/Electrical Sensors/Current Sensor
  I_x : fl_lib/Electrical/Electrical Sensors/Current Sensor
  L_b : fl_lib/Electrical/Electrical Elements/Inductor  l=TB.C.L H  r=TB.C.RL Ohm  g=1e-9 1/Ohm  i_specify=off  i_priority=None  i=0 A  i_nominal_specify=off  i_nominal_value=1  i_nominal_unit=A  v_specify=off  v_priority=None  v=0 V  v_nominal_specify=off  v_nominal_value=1  v_nominal_unit=V  i_L_specify=on  i_L_priority=High  i_L=TB.x0(1) A  i_L_nominal_specify=off  i_L_nominal_value=1  i_L_nominal_unit=A
  L_m : fl_lib/Electrical/Electrical Elements/Inductor  l=TB.C.Lm H  r=0 Ohm  g=1e-9 1/Ohm  i_specify=off  i_priority=None  i=0 A  i_nominal_specify=off  i_nominal_value=1  i_nominal_unit=A  v_specify=off  v_priority=None  v=0 V  v_nominal_specify=off  v_nominal_value=1  v_nominal_unit=V  i_L_specify=on  i_L_priority=High  i_L=0 A  i_L_nominal_specify=off  i_L_nominal_value=1  i_L_nominal_unit=A
  L_r1 : fl_lib/Electrical/Electrical Elements/Inductor  l=TB.C.Lr1 H  r=TB.C.Rw1 Ohm  g=1e-9 1/Ohm  i_specify=off  i_priority=None  i=0 A  i_nominal_specify=off  i_nominal_value=1  i_nominal_unit=A  v_specify=off  v_priority=None  v=0 V  v_nominal_specify=off  v_nominal_value=1  v_nominal_unit=V  i_L_specify=on  i_L_priority=High  i_L=0 A  i_L_nominal_specify=off  i_L_nominal_value=1  i_L_nominal_unit=A
  L_r2 : fl_lib/Electrical/Electrical Elements/Inductor  l=TB.C.Lr2 H  r=TB.C.Rw2 Ohm  g=1e-9 1/Ohm  i_specify=off  i_priority=None  i=0 A  i_nominal_specify=off  i_nominal_value=1  i_nominal_unit=A  v_specify=off  v_priority=None  v=0 V  v_nominal_specify=off  v_nominal_value=1  v_nominal_unit=V  i_L_specify=on  i_L_priority=High  i_L=0 A  i_L_nominal_specify=off  i_L_nominal_value=1  i_L_nominal_unit=A
  Primary_Bridge : Subsystem
  SB_H_high : Subsystem  mask(PRISM-Hub switch cell){Ron=TB.SB.Ron, Goff=TB.SB.Goff, Vf=TB.SB.Vf, Rd=TB.SB.Rd, Goffd=TB.SB.Goffd, Coss=TB.SB.Coss}
      mask prompts: Ron "도통 저항 R_on [Ohm]"; Goff "차단 컨덕턴스 G_off [S]"; Vf "다이오드 순방향 전압 Vf [V]"; Rd "다이오드 도통 저항 R_d [Ohm]"; Goffd "다이오드 차단 컨덕턴스 [S]"; Coss "출력용량 C_oss [F]"
      mask help: 전력 반도체 스위치 셀 SB_H. 게이트 태그 gS_BH.
      settings: AttributesFormatString=gate: gS_BH
      mask Display:
      | plot([0.50 0.50 ],[0.95 0.65 ],[0.50 0.74 ],[0.65 0.35 ],[0.50 0.50 ],[0.35 0.05 ]);
      | plot([0.50 0.20 0.20 ],[0.80 0.80 0.58 ],[0.20 0.20 0.50 ],[0.42 0.20 0.20 ]);
      | plot([0.20 0.10 0.30 0.20 ],[0.58 0.42 0.42 0.58 ],[0.10 0.30 ],[0.58 0.58 ]);
      | port_label('LConn',1,'D');
      | port_label('RConn',1,'S');
  SB_L_low : Subsystem  mask(PRISM-Hub switch cell){Ron=TB.SB.Ron, Goff=TB.SB.Goff, Vf=TB.SB.Vf, Rd=TB.SB.Rd, Goffd=TB.SB.Goffd, Coss=TB.SB.Coss}
      mask prompts: Ron "도통 저항 R_on [Ohm]"; Goff "차단 컨덕턴스 G_off [S]"; Vf "다이오드 순방향 전압 Vf [V]"; Rd "다이오드 도통 저항 R_d [Ohm]"; Goffd "다이오드 차단 컨덕턴스 [S]"; Coss "출력용량 C_oss [F]"
      mask help: 전력 반도체 스위치 셀 SB_L. 게이트 태그 gS_BL.
      settings: AttributesFormatString=gate: gS_BL
      mask Display:
      | plot([0.50 0.50 ],[0.95 0.65 ],[0.50 0.74 ],[0.65 0.35 ],[0.50 0.50 ],[0.35 0.05 ]);
      | plot([0.50 0.20 0.20 ],[0.80 0.80 0.58 ],[0.20 0.20 0.50 ],[0.42 0.20 0.20 ]);
      | plot([0.20 0.10 0.30 0.20 ],[0.58 0.42 0.42 0.58 ],[0.10 0.30 ],[0.58 0.58 ]);
      | port_label('LConn',1,'D');
      | port_label('RConn',1,'S');
  Secondary_Bridge : Subsystem
  V_Cr1 : fl_lib/Electrical/Electrical Sensors/Voltage Sensor
  V_I : fl_lib/Electrical/Electrical Sensors/Voltage Sensor
  V_leg1 : fl_lib/Electrical/Electrical Sensors/Voltage Sensor
  V_legs1 : fl_lib/Electrical/Electrical Sensors/Voltage Sensor
  V_swb : fl_lib/Electrical/Electrical Sensors/Voltage Sensor
  Xfmr_n1 : fl_lib/Electrical/Electrical Elements/Ideal Transformer  n=TB.C.n  i1_specify=off  i1_priority=None  i1=0 A  i1_nominal_specify=off  i1_nominal_value=1  i1_nominal_unit=A  v1_specify=off  v1_priority=None  v1=0 V  v1_nominal_specify=off  v1_nominal_value=1  v1_nominal_unit=V  i2_specify=off  i2_priority=None  i2=0 A  i2_nominal_specify=off  i2_nominal_value=1  i2_nominal_unit=A  v2_specify=off  v2_priority=None  v2=0 V  v2_nominal_specify=off  v2_nominal_value=1  v2_nominal_unit=V
  iL_PS2SL : nesl_utility/PS-Simulink Converter  PhysicalDomain=network_engine_domain  SubClassName=ps_output  LeftPortType=input  RightPortType=output  PseudoPeriodic=off  Frequencies=[]  VectorFormat=inherit  Unit=inherit  AffineConversion=off
  im_PS2SL : nesl_utility/PS-Simulink Converter  PhysicalDomain=network_engine_domain  SubClassName=ps_output  LeftPortType=input  RightPortType=output  PseudoPeriodic=off  Frequencies=[]  VectorFormat=inherit  Unit=inherit  AffineConversion=off
  ir1_PS2SL : nesl_utility/PS-Simulink Converter  PhysicalDomain=network_engine_domain  SubClassName=ps_output  LeftPortType=input  RightPortType=output  PseudoPeriodic=off  Frequencies=[]  VectorFormat=inherit  Unit=inherit  AffineConversion=off
  ir2_PS2SL : nesl_utility/PS-Simulink Converter  PhysicalDomain=network_engine_domain  SubClassName=ps_output  LeftPortType=input  RightPortType=output  PseudoPeriodic=off  Frequencies=[]  VectorFormat=inherit  Unit=inherit  AffineConversion=off
  ix_PS2SL : nesl_utility/PS-Simulink Converter  PhysicalDomain=network_engine_domain  SubClassName=ps_output  LeftPortType=input  RightPortType=output  PseudoPeriodic=off  Frequencies=[]  VectorFormat=inherit  Unit=inherit  AffineConversion=off
  vI_PS2SL : nesl_utility/PS-Simulink Converter  PhysicalDomain=network_engine_domain  SubClassName=ps_output  LeftPortType=input  RightPortType=output  PseudoPeriodic=off  Frequencies=[]  VectorFormat=inherit  Unit=inherit  AffineConversion=off
  vcr1_PS2SL : nesl_utility/PS-Simulink Converter  PhysicalDomain=network_engine_domain  SubClassName=ps_output  LeftPortType=input  RightPortType=output  PseudoPeriodic=off  Frequencies=[]  VectorFormat=inherit  Unit=inherit  AffineConversion=off
  vleg1_PS2SL : nesl_utility/PS-Simulink Converter  PhysicalDomain=network_engine_domain  SubClassName=ps_output  LeftPortType=input  RightPortType=output  PseudoPeriodic=off  Frequencies=[]  VectorFormat=inherit  Unit=inherit  AffineConversion=off
  vlegs1_PS2SL : nesl_utility/PS-Simulink Converter  PhysicalDomain=network_engine_domain  SubClassName=ps_output  LeftPortType=input  RightPortType=output  PseudoPeriodic=off  Frequencies=[]  VectorFormat=inherit  Unit=inherit  AffineConversion=off
  vswb_PS2SL : nesl_utility/PS-Simulink Converter  PhysicalDomain=network_engine_domain  SubClassName=ps_output  LeftPortType=input  RightPortType=output  PseudoPeriodic=off  Frequencies=[]  VectorFormat=inherit  Unit=inherit  AffineConversion=off
  DC_P : PMIOPort  Side=Left
  DC_N : PMIOPort  Port=2  Side=Left
  VO_P : PMIOPort  Port=3  Side=Right
  VO_N : PMIOPort  Port=4  Side=Right
  tag scope: iL=global, im=global, ir1=global, ir2=global, ix=global, vI=global, vcr1=global, vleg1=global, vlegs1=global, vswb=global
  wires:
  iL_PS2SL/1 -> [iL]
  vI_PS2SL/1 -> [vI]
  vswb_PS2SL/1 -> [vswb]
  ir1_PS2SL/1 -> [ir1]
  im_PS2SL/1 -> [im]
  ir2_PS2SL/1 -> [ir2]
  ix_PS2SL/1 -> [ix]
  vcr1_PS2SL/1 -> [vcr1]
  vleg1_PS2SL/1 -> [vleg1]
  vlegs1_PS2SL/1 -> [vlegs1]
  connections:
  SB_H_high/LConn1 -- DC_P/RConn1
  SB_L_low/LConn1 -- SB_H_high/RConn1 -- L_b/LConn1 -- V_swb/LConn1
  SB_L_low/RConn1 -- C_I/RConn1 -- V_I/RConn2 -- V_swb/RConn2 -- Primary_Bridge/LConn2 -- DC_N/RConn1 -- V_leg1/RConn2
  L_b/RConn1 -- I_L/LConn1
  I_L/RConn2 -- V_I/LConn1 -- C_I/LConn1 -- Primary_Bridge/LConn1
  C_r1/LConn1 -- Primary_Bridge/RConn1 -- V_leg1/LConn1 -- V_Cr1/LConn1
  L_r1/LConn1 -- C_r1/RConn1 -- V_Cr1/RConn2
  L_r1/RConn1 -- I_r1/LConn1
  Xfmr_n1/LConn1 -- I_r1/RConn2 -- I_m/LConn1
  Primary_Bridge/RConn2 -- Xfmr_n1/LConn2 -- L_m/RConn1
  I_m/RConn2 -- L_m/LConn1
  Xfmr_n1/RConn1 -- L_r2/LConn1
  L_r2/RConn1 -- C_r2/LConn1
  C_r2/RConn1 -- I_r2/LConn1
  Secondary_Bridge/RConn1 -- I_r2/RConn2 -- V_legs1/LConn1
  Xfmr_n1/RConn2 -- Secondary_Bridge/RConn2
  Secondary_Bridge/LConn1 -- I_x/LConn1
  C_o/LConn1 -- I_x/RConn2 -- VO_P/RConn1
  Secondary_Bridge/LConn2 -- VO_N/RConn1 -- V_legs1/RConn2 -- C_o/RConn1 -- GND_secondary/LConn1
  I_L/RConn1 -- iL_PS2SL/LConn1
  V_I/RConn1 -- vI_PS2SL/LConn1
  V_swb/RConn1 -- vswb_PS2SL/LConn1
  I_r1/RConn1 -- ir1_PS2SL/LConn1
  I_m/RConn1 -- im_PS2SL/LConn1
  I_r2/RConn1 -- ir2_PS2SL/LConn1
  I_x/RConn1 -- ix_PS2SL/LConn1
  V_Cr1/RConn1 -- vcr1_PS2SL/LConn1
  V_leg1/RConn1 -- vleg1_PS2SL/LConn1
  V_legs1/RConn1 -- vlegs1_PS2SL/LConn1

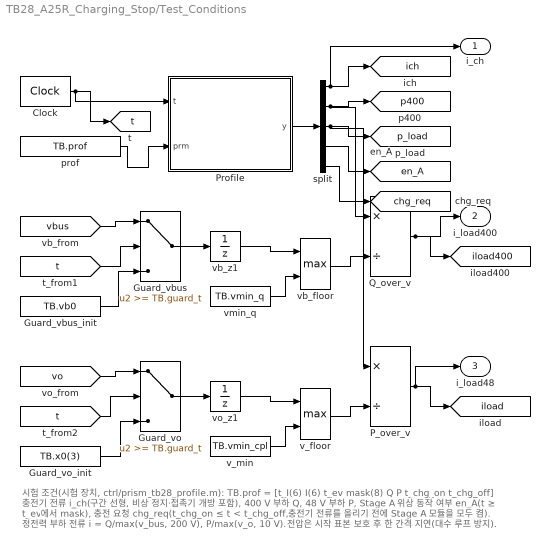
== system TB28_A25R_Charging_Stop/Test_Conditions ==
  note: 시험 조건(시험 장치, ctrl/prism_tb28_profile.m): TB.prof = [t_I(6) I(6) t_ev mask(8) Q P t_chg_on t_chg_off]
      | 충전기 전류 i_ch(구간 선형, 비상 정지·접촉기 개방 포함), 400 V 부하 Q, 48 V 부하 P, Stage A 위상 동작 여부 en_A(t ≥ t_ev에서 mask),
      | 충전 요청 chg_req(t_chg_on ≤ t < t_chg_off, 충전기 전류를 올리기 전에 Stage A 모듈을 모두 켬).
      | 정전력 부하 전류 i = Q/max(v_bus, 200 V), P/max(v_o, 10 V). 전압은 시작 표본 보호 후 한 간격 지연(대수 루프 방지).
  Clock : DigitalClock  SampleTime=TB.dt
  Guard_vbus : Switch  Threshold=TB.guard_t  SaturateOnIntegerOverflow=off  InputSameDT=off
  Guard_vbus_init : Constant  Value=TB.vb0
  Guard_vo : Switch  Threshold=TB.guard_t  SaturateOnIntegerOverflow=off  InputSameDT=off
  Guard_vo_init : Constant  Value=TB.x0(3)
  P_over_v : Product  Inputs=*/
  Profile : MATLAB Function  TreatAsAtomicUnit=on
  Q_over_v : Product  Inputs=*/
  prof : Constant  Value=TB.prof
  split : Demux  Outputs=[1 1 1 8 1]
  v_floor : MinMax  Function=max  Inputs=2
  v_min : Constant  Value=TB.vmin_cpl
  vb_floor : MinMax  Function=max  Inputs=2
  vb_z1 : UnitDelay  SampleTime=TB.dt  HasFrameUpgradeWarning=on
  vmin_q : Constant  Value=TB.vmin_q
  vo_z1 : UnitDelay  SampleTime=TB.dt  HasFrameUpgradeWarning=on
  i_ch : Outport
  i_load400 : Outport  Port=2
  i_load48 : Outport  Port=3
  tag scope: chg_req=global, en_A=global, ich=global, iload400=global, iload=global, p400=global, p_load=global, t=global
  wires:
  Clock/1 -> [t], Profile/1(t)
  prof/1 -> Profile/2(prm)
  Profile/1(y) -> split/1
  split/1 -> [ich], i_ch/1
  split/2 -> [p400], Q_over_v/1
  split/3 -> [p_load], P_over_v/1
  split/4 -> [en_A]
  split/5 -> [chg_req]
  Guard_vbus_init/1 -> Guard_vbus/3
  [vbus] -> Guard_vbus/1
  [t] -> Guard_vbus/2
  Guard_vbus/1 -> vb_z1/1
  vb_z1/1 -> vb_floor/1
  vmin_q/1 -> vb_floor/2
  vb_floor/1 -> Q_over_v/2
  Q_over_v/1 -> [iload400], i_load400/1
  Guard_vo_init/1 -> Guard_vo/3
  [vo] -> Guard_vo/1
  [t] -> Guard_vo/2
  Guard_vo/1 -> vo_z1/1
  vo_z1/1 -> v_floor/1
  v_min/1 -> v_floor/2
  v_floor/1 -> P_over_v/2
  P_over_v/1 -> [iload], i_load48/1
